simulink model "gofa_robot"  (R2023a)
settings: Solver=FixedStepAuto  StartTime=0.0  StopTime=11  FixedStep=0.001  RelTol=1e-3
undefined symbols (not defined in the file or in its folder): X, Y, Z
libraries: sm_lib x58, nesl_utility x10, slpidlib x3
(part 7 of 7)

== matlab function gofa_robot/inverse_Jacobian1 ==
  data: output_djoint_value output; dx input; det_J output; dy input; dz input; d_alpha input; d_beta input; d_gamma input; joint_value input
% function [dq1,dq2,dq3,dq4,dq5,dq6] = fcn(dx,dy,dz,d_alpha,d_beta,d_gamma, joint_value)
%function [output_joint_value,output_djoint_value,det_J]  = inverse_Jacobian(dx,dy,dz,d_alpha,d_beta,d_gamma, joint_value)
function [output_djoint_value,det_J]  = inverse_Jacobian(dx,dy,dz,d_alpha,d_beta,d_gamma, joint_value)
% persistent theta1 theta2 theta3 theta4 theta5 theta6
% if isempty(theta1)
%     theta1 =  1e-5;
%     theta2 =  1e-5;
%     theta3 =  1e-5;
%     theta4 =  1e-5;
%     theta5 =  1e-5;
%     theta6 =  1e-5;    
% end

if (length(joint_value)>1)
    q1 = joint_value(1);
    q2 = joint_value(2);
    q3 = joint_value(3);
    q4 = joint_value(4);
    q5 = joint_value(5);
    q6 = joint_value(6);
else
    q1 =  1e-5;
    q2 =  1e-5;
    q3 =  1e-5;
    q4 =  1e-5;
    q5 =  1e-5;
    q6 =  1e-5;
end

J = zeros(6,6);
J(1,1)= (551421093602387721*cos(q1)*cos(q2))/20282409603651670423947251286016000 - (15367999408544611283610854417045082301222635242944759808457209068371609267073198931*cos(q1))/533996758980227520598755426542388028650676130589163192486760401955554931445160137505740521734144000 - (501743517602172611*cos(q1)*cos(q4))/81129638414606681695789005144064000 + (3093548567763867359251342063207821441907716257110899757329320000341*sin(q3)*((81129638414606676728031405122553*cos(q1 - q2))/2 - (81129638414606686663546605165575*cos(q1 + q2))/2))/533996758980227520598755426542388028650676130589163192486760401955554931445160137505740521734144000 - (3093548567763867359251342063207821441907716257110899757329320000341*cos(q3)*((81129638414606676728031405122553*sin(q1 - q2))/2 + (81129638414606686663546605165575*sin(q1 + q2))/2))/533996758980227520598755426542388028650676130589163192486760401955554931445160137505740521734144000 - (111*sin(q1)*sin(q2))/250 - (11*sin(q3)*((81129638414606676728031405122553*sin(q1 - q2))/2 + (81129638414606686663546605165575*sin(q1 + q2))/2))/8112963841460668169578900514406400 - (101*cos(q5)*((81129638414606686663546605165575*sin(q1 + q2 + q3))/162259276829213363391578010288128 - (81129638414606676728031405122553*sin(q2 - q1 + q3))/162259276829213363391578010288128 + (4967757600021511*cos(q1))/81129638414606681695789005144064))/1000 - (sin(q5)*(81129638414606686663546605165575*sin(q1 + q2 + q3) - 81129638414606676728031405122553*sin(q2 - q1 + q3) + 9935515200043022*cos(q1)))/2028240960365167042394725128601600 - (501743517602172611*cos(q5)*((sin(q4)*(81129638414606686663546605165575*cos(q1 + q2 + q3) - 81129638414606676728031405122553*cos(q2 - q1 + q3)))/162259276829213363391578010288128 - cos(q1)*cos(q4) + (4967757600021511*cos(q4)*((81129638414606686663546605165575*sin(q1 + q2 + q3))/162259276829213363391578010288128 - (81129638414606676728031405122553*sin(q2 - q1 + q3))/162259276829213363391578010288128))/81129638414606681695789005144064))/81129638414606681695789005144064000 + (2*cos(q5)*(cos(q1)*sin(q4) - (4967757600021511*sin(q4)*((81129638414606686663546605165575*sin(q1 + q2 + q3))/162259276829213363391578010288128 - (81129638414606676728031405122553*sin(q2 - q1 + q3))/162259276829213363391578010288128))/81129638414606681695789005144064 + cos(q4)*((81129638414606686663546605165575*cos(q1 + q2 + q3))/162259276829213363391578010288128 - (81129638414606676728031405122553*cos(q2 - q1 + q3))/162259276829213363391578010288128)))/25 - (4967757600021511*sin(q5)*((sin(q4)*(81129638414606686663546605165575*cos(q1 + q2 + q3) - 81129638414606676728031405122553*cos(q2 - q1 + q3)))/162259276829213363391578010288128 - cos(q1)*cos(q4) + (4967757600021511*cos(q4)*((81129638414606686663546605165575*sin(q1 + q2 + q3))/162259276829213363391578010288128 - (81129638414606676728031405122553*sin(q2 - q1 + q3))/162259276829213363391578010288128))/81129638414606681695789005144064))/1014120480182583521197362564300800 - (101*sin(q5)*(cos(q1)*sin(q4) - (4967757600021511*sin(q4)*((81129638414606686663546605165575*sin(q1 + q2 + q3))/162259276829213363391578010288128 - (81129638414606676728031405122553*sin(q2 - q1 + q3))/162259276829213363391578010288128))/81129638414606681695789005144064 + cos(q4)*((81129638414606686663546605165575*cos(q1 + q2 + q3))/162259276829213363391578010288128 - (81129638414606676728031405122553*cos(q2 - q1 + q3))/162259276829213363391578010288128)))/1000 + (501743517602172611*sin(q4)*((81129638414606686663546605165575*cos(q1 + q2 + q3))/162259276829213363391578010288128 - (81129638414606676728031405122553*cos(q2 - q1 + q3))/162259276829213363391578010288128))/81129638414606681695789005144064000 - (11*cos(q3)*((81129638414606676728031405122553*cos(q1 - q2))/2 - (81129638414606686663546605165575*cos(q1 + q2))/2))/8112963841460668169578900514406400 + (2492540172829719769614233935035221*cos(q4)*((81129638414606686663546605165575*sin(q1 + q2 + q3))/162259276829213363391578010288128 - (81129638414606676728031405122553*sin(q2 - q1 + q3))/162259276829213363391578010288128))/6582018229284824168619876730229402019930943462534319453394436096000;
J(1,2)=(111*cos(q1)*cos(q2))/250 - (3093548567763867359251342063207821441907716257110899757329320000341*sin(q3)*((81129638414606676728031405122553*cos(q1 - q2))/2 + (81129638414606686663546605165575*cos(q1 + q2))/2))/533996758980227520598755426542388028650676130589163192486760401955554931445160137505740521734144000 - (sin(q5)*(81129638414606686663546605165575*sin(q1 + q2 + q3) + 81129638414606676728031405122553*sin(q2 - q1 + q3)))/2028240960365167042394725128601600 + (3093548567763867359251342063207821441907716257110899757329320000341*cos(q3)*((81129638414606676728031405122553*sin(q1 - q2))/2 - (81129638414606686663546605165575*sin(q1 + q2))/2))/533996758980227520598755426542388028650676130589163192486760401955554931445160137505740521734144000 - (551421093602387721*sin(q1)*sin(q2))/20282409603651670423947251286016000 + (11*sin(q3)*((81129638414606676728031405122553*sin(q1 - q2))/2 - (81129638414606686663546605165575*sin(q1 + q2))/2))/8112963841460668169578900514406400 - (501743517602172611*cos(q5)*(sin(q4)*((81129638414606686663546605165575*cos(q1 + q2 + q3))/162259276829213363391578010288128 + (81129638414606676728031405122553*cos(q2 - q1 + q3))/162259276829213363391578010288128) + (4967757600021511*cos(q4)*((81129638414606686663546605165575*sin(q1 + q2 + q3))/162259276829213363391578010288128 + (81129638414606676728031405122553*sin(q2 - q1 + q3))/162259276829213363391578010288128))/81129638414606681695789005144064))/81129638414606681695789005144064000 - (2*cos(q5)*((4967757600021511*sin(q4)*((81129638414606686663546605165575*sin(q1 + q2 + q3))/162259276829213363391578010288128 + (81129638414606676728031405122553*sin(q2 - q1 + q3))/162259276829213363391578010288128))/81129638414606681695789005144064 - cos(q4)*((81129638414606686663546605165575*cos(q1 + q2 + q3))/162259276829213363391578010288128 + (81129638414606676728031405122553*cos(q2 - q1 + q3))/162259276829213363391578010288128)))/25 - (4967757600021511*sin(q5)*(sin(q4)*((81129638414606686663546605165575*cos(q1 + q2 + q3))/162259276829213363391578010288128 + (81129638414606676728031405122553*cos(q2 - q1 + q3))/162259276829213363391578010288128) + (4967757600021511*cos(q4)*((81129638414606686663546605165575*sin(q1 + q2 + q3))/162259276829213363391578010288128 + (81129638414606676728031405122553*sin(q2 - q1 + q3))/162259276829213363391578010288128))/81129638414606681695789005144064))/1014120480182583521197362564300800 + (101*sin(q5)*((4967757600021511*sin(q4)*((81129638414606686663546605165575*sin(q1 + q2 + q3))/162259276829213363391578010288128 + (81129638414606676728031405122553*sin(q2 - q1 + q3))/162259276829213363391578010288128))/81129638414606681695789005144064 - cos(q4)*((81129638414606686663546605165575*cos(q1 + q2 + q3))/162259276829213363391578010288128 + (81129638414606676728031405122553*cos(q2 - q1 + q3))/162259276829213363391578010288128)))/1000 + (501743517602172611*sin(q4)*((81129638414606686663546605165575*cos(q1 + q2 + q3))/162259276829213363391578010288128 + (81129638414606676728031405122553*cos(q2 - q1 + q3))/162259276829213363391578010288128))/81129638414606681695789005144064000 + (11*cos(q3)*((81129638414606676728031405122553*cos(q1 - q2))/2 + (81129638414606686663546605165575*cos(q1 + q2))/2))/8112963841460668169578900514406400 + (2492540172829719769614233935035221*cos(q4)*((81129638414606686663546605165575*sin(q1 + q2 + q3))/162259276829213363391578010288128 + (81129638414606676728031405122553*sin(q2 - q1 + q3))/162259276829213363391578010288128))/6582018229284824168619876730229402019930943462534319453394436096000 - (101*cos(q5)*((81129638414606686663546605165575*sin(q1 + q2 + q3))/162259276829213363391578010288128 + (81129638414606676728031405122553*sin(q2 - q1 + q3))/162259276829213363391578010288128))/1000;
J(1,3)= (3093548567763867359251342063207821441907716257110899757329320000341*cos(q3)*((81129638414606676728031405122553*sin(q1 - q2))/2 - (81129638414606686663546605165575*sin(q1 + q2))/2))/533996758980227520598755426542388028650676130589163192486760401955554931445160137505740521734144000 - (sin(q5)*(81129638414606686663546605165575*sin(q1 + q2 + q3) + 81129638414606676728031405122553*sin(q2 - q1 + q3)))/2028240960365167042394725128601600 - (3093548567763867359251342063207821441907716257110899757329320000341*sin(q3)*((81129638414606676728031405122553*cos(q1 - q2))/2 + (81129638414606686663546605165575*cos(q1 + q2))/2))/533996758980227520598755426542388028650676130589163192486760401955554931445160137505740521734144000 + (11*sin(q3)*((81129638414606676728031405122553*sin(q1 - q2))/2 - (81129638414606686663546605165575*sin(q1 + q2))/2))/8112963841460668169578900514406400 - (501743517602172611*cos(q5)*(sin(q4)*((81129638414606686663546605165575*cos(q1 + q2 + q3))/162259276829213363391578010288128 + (81129638414606676728031405122553*cos(q2 - q1 + q3))/162259276829213363391578010288128) + (4967757600021511*cos(q4)*((81129638414606686663546605165575*sin(q1 + q2 + q3))/162259276829213363391578010288128 + (81129638414606676728031405122553*sin(q2 - q1 + q3))/162259276829213363391578010288128))/81129638414606681695789005144064))/81129638414606681695789005144064000 - (2*cos(q5)*((4967757600021511*sin(q4)*((81129638414606686663546605165575*sin(q1 + q2 + q3))/162259276829213363391578010288128 + (81129638414606676728031405122553*sin(q2 - q1 + q3))/162259276829213363391578010288128))/81129638414606681695789005144064 - cos(q4)*((81129638414606686663546605165575*cos(q1 + q2 + q3))/162259276829213363391578010288128 + (81129638414606676728031405122553*cos(q2 - q1 + q3))/162259276829213363391578010288128)))/25 - (4967757600021511*sin(q5)*(sin(q4)*((81129638414606686663546605165575*cos(q1 + q2 + q3))/162259276829213363391578010288128 + (81129638414606676728031405122553*cos(q2 - q1 + q3))/162259276829213363391578010288128) + (4967757600021511*cos(q4)*((81129638414606686663546605165575*sin(q1 + q2 + q3))/162259276829213363391578010288128 + (81129638414606676728031405122553*sin(q2 - q1 + q3))/162259276829213363391578010288128))/81129638414606681695789005144064))/1014120480182583521197362564300800 + (101*sin(q5)*((4967757600021511*sin(q4)*((81129638414606686663546605165575*sin(q1 + q2 + q3))/162259276829213363391578010288128 + (81129638414606676728031405122553*sin(q2 - q1 + q3))/162259276829213363391578010288128))/81129638414606681695789005144064 - cos(q4)*((81129638414606686663546605165575*cos(q1 + q2 + q3))/162259276829213363391578010288128 + (81129638414606676728031405122553*cos(q2 - q1 + q3))/162259276829213363391578010288128)))/1000 + (501743517602172611*sin(q4)*((81129638414606686663546605165575*cos(q1 + q2 + q3))/162259276829213363391578010288128 + (81129638414606676728031405122553*cos(q2 - q1 + q3))/162259276829213363391578010288128))/81129638414606681695789005144064000 + (11*cos(q3)*((81129638414606676728031405122553*cos(q1 - q2))/2 + (81129638414606686663546605165575*cos(q1 + q2))/2))/8112963841460668169578900514406400 + (2492540172829719769614233935035221*cos(q4)*((81129638414606686663546605165575*sin(q1 + q2 + q3))/162259276829213363391578010288128 + (81129638414606676728031405122553*sin(q2 - q1 + q3))/162259276829213363391578010288128))/6582018229284824168619876730229402019930943462534319453394436096000 - (101*cos(q5)*((81129638414606686663546605165575*sin(q1 + q2 + q3))/162259276829213363391578010288128 + (81129638414606676728031405122553*sin(q2 - q1 + q3))/162259276829213363391578010288128))/1000;
J(1,4)=(501743517602172611*sin(q1)*sin(q4))/81129638414606681695789005144064000 + (2*cos(q5)*(cos(q4)*sin(q1) - sin(q4)*((81129638414606686663546605165575*sin(q1 + q2 + q3))/162259276829213363391578010288128 + (81129638414606676728031405122553*sin(q2 - q1 + q3))/162259276829213363391578010288128) + (4967757600021511*cos(q4)*((81129638414606686663546605165575*cos(q1 + q2 + q3))/162259276829213363391578010288128 + (81129638414606676728031405122553*cos(q2 - q1 + q3))/162259276829213363391578010288128))/81129638414606681695789005144064))/25 - (501743517602172611*cos(q5)*(sin(q1)*sin(q4) + (4967757600021511*sin(q4)*((81129638414606686663546605165575*cos(q1 + q2 + q3))/162259276829213363391578010288128 + (81129638414606676728031405122553*cos(q2 - q1 + q3))/162259276829213363391578010288128))/81129638414606681695789005144064 + cos(q4)*((81129638414606686663546605165575*sin(q1 + q2 + q3))/162259276829213363391578010288128 + (81129638414606676728031405122553*sin(q2 - q1 + q3))/162259276829213363391578010288128)))/81129638414606681695789005144064000 - (101*sin(q5)*(cos(q4)*sin(q1) - sin(q4)*((81129638414606686663546605165575*sin(q1 + q2 + q3))/162259276829213363391578010288128 + (81129638414606676728031405122553*sin(q2 - q1 + q3))/162259276829213363391578010288128) + (4967757600021511*cos(q4)*((81129638414606686663546605165575*cos(q1 + q2 + q3))/162259276829213363391578010288128 + (81129638414606676728031405122553*cos(q2 - q1 + q3))/162259276829213363391578010288128))/81129638414606681695789005144064))/1000 - (4967757600021511*sin(q5)*(sin(q1)*sin(q4) + (4967757600021511*sin(q4)*((81129638414606686663546605165575*cos(q1 + q2 + q3))/162259276829213363391578010288128 + (81129638414606676728031405122553*cos(q2 - q1 + q3))/162259276829213363391578010288128))/81129638414606681695789005144064 + cos(q4)*((81129638414606686663546605165575*sin(q1 + q2 + q3))/162259276829213363391578010288128 + (81129638414606676728031405122553*sin(q2 - q1 + q3))/162259276829213363391578010288128)))/1014120480182583521197362564300800 + (2492540172829719769614233935035221*sin(q4)*((81129638414606686663546605165575*cos(q1 + q2 + q3))/162259276829213363391578010288128 + (81129638414606676728031405122553*cos(q2 - q1 + q3))/162259276829213363391578010288128))/6582018229284824168619876730229402019930943462534319453394436096000 + (501743517602172611*cos(q4)*((81129638414606686663546605165575*sin(q1 + q2 + q3))/162259276829213363391578010288128 + (81129638414606676728031405122553*sin(q2 - q1 + q3))/162259276829213363391578010288128))/81129638414606681695789005144064000;
J(1,5)=(cos(q5)*(81129638414606686663546605165575*cos(q1 + q2 + q3) + 81129638414606676728031405122553*cos(q2 - q1 + q3) - 9935515200043022*sin(q1)))/2028240960365167042394725128601600 - (101*sin(q5)*((81129638414606686663546605165575*cos(q1 + q2 + q3))/162259276829213363391578010288128 + (81129638414606676728031405122553*cos(q2 - q1 + q3))/162259276829213363391578010288128 - (4967757600021511*sin(q1))/81129638414606681695789005144064))/1000 + (4967757600021511*cos(q5)*(cos(q4)*sin(q1) - sin(q4)*((81129638414606686663546605165575*sin(q1 + q2 + q3))/162259276829213363391578010288128 + (81129638414606676728031405122553*sin(q2 - q1 + q3))/162259276829213363391578010288128) + (4967757600021511*cos(q4)*((81129638414606686663546605165575*cos(q1 + q2 + q3))/162259276829213363391578010288128 + (81129638414606676728031405122553*cos(q2 - q1 + q3))/162259276829213363391578010288128))/81129638414606681695789005144064))/1014120480182583521197362564300800 - (101*cos(q5)*(sin(q1)*sin(q4) + (4967757600021511*sin(q4)*((81129638414606686663546605165575*cos(q1 + q2 + q3))/162259276829213363391578010288128 + (81129638414606676728031405122553*cos(q2 - q1 + q3))/162259276829213363391578010288128))/81129638414606681695789005144064 + cos(q4)*((81129638414606686663546605165575*sin(q1 + q2 + q3))/162259276829213363391578010288128 + (81129638414606676728031405122553*sin(q2 - q1 + q3))/162259276829213363391578010288128)))/1000 - (501743517602172611*sin(q5)*(cos(q4)*sin(q1) - sin(q4)*((81129638414606686663546605165575*sin(q1 + q2 + q3))/162259276829213363391578010288128 + (81129638414606676728031405122553*sin(q2 - q1 + q3))/162259276829213363391578010288128) + (4967757600021511*cos(q4)*((81129638414606686663546605165575*cos(q1 + q2 + q3))/162259276829213363391578010288128 + (81129638414606676728031405122553*cos(q2 - q1 + q3))/162259276829213363391578010288128))/81129638414606681695789005144064))/81129638414606681695789005144064000 - (2*sin(q5)*(sin(q1)*sin(q4) + (4967757600021511*sin(q4)*((81129638414606686663546605165575*cos(q1 + q2 + q3))/162259276829213363391578010288128 + (81129638414606676728031405122553*cos(q2 - q1 + q3))/162259276829213363391578010288128))/81129638414606681695789005144064 + cos(q4)*((81129638414606686663546605165575*sin(q1 + q2 + q3))/162259276829213363391578010288128 + (81129638414606676728031405122553*sin(q2 - q1 + q3))/162259276829213363391578010288128)))/25;
J(1,6)= 0;

J(2,1)=(11*sin(q3)*((81129638414606676728031405122553*cos(q1 - q2))/2 + (81129638414606686663546605165575*cos(q1 + q2))/2))/8112963841460668169578900514406400 - (15367999408544611283610854417045082301222635242944759808457209068371609267073198931*sin(q1))/533996758980227520598755426542388028650676130589163192486760401955554931445160137505740521734144000 + (501743517602172611*sin(q4)*((81129638414606686663546605165575*sin(q1 + q2 + q3))/162259276829213363391578010288128 + (81129638414606676728031405122553*sin(q2 - q1 + q3))/162259276829213363391578010288128))/81129638414606681695789005144064000 + (111*cos(q1)*sin(q2))/250 + (551421093602387721*cos(q2)*sin(q1))/20282409603651670423947251286016000 - (501743517602172611*cos(q4)*sin(q1))/81129638414606681695789005144064000 - (11*cos(q3)*((81129638414606676728031405122553*sin(q1 - q2))/2 - (81129638414606686663546605165575*sin(q1 + q2))/2))/8112963841460668169578900514406400 + (3093548567763867359251342063207821441907716257110899757329320000341*sin(q3)*((81129638414606676728031405122553*sin(q1 - q2))/2 - (81129638414606686663546605165575*sin(q1 + q2))/2))/533996758980227520598755426542388028650676130589163192486760401955554931445160137505740521734144000 + (101*cos(q5)*((81129638414606686663546605165575*cos(q1 + q2 + q3))/162259276829213363391578010288128 + (81129638414606676728031405122553*cos(q2 - q1 + q3))/162259276829213363391578010288128 - (4967757600021511*sin(q1))/81129638414606681695789005144064))/1000 + (sin(q5)*(81129638414606686663546605165575*cos(q1 + q2 + q3) + 81129638414606676728031405122553*cos(q2 - q1 + q3) - 9935515200043022*sin(q1)))/2028240960365167042394725128601600 + (501743517602172611*cos(q5)*(cos(q4)*sin(q1) - sin(q4)*((81129638414606686663546605165575*sin(q1 + q2 + q3))/162259276829213363391578010288128 + (81129638414606676728031405122553*sin(q2 - q1 + q3))/162259276829213363391578010288128) + (4967757600021511*cos(q4)*((81129638414606686663546605165575*cos(q1 + q2 + q3))/162259276829213363391578010288128 + (81129638414606676728031405122553*cos(q2 - q1 + q3))/162259276829213363391578010288128))/81129638414606681695789005144064))/81129638414606681695789005144064000 + (2*cos(q5)*(sin(q1)*sin(q4) + (4967757600021511*sin(q4)*((81129638414606686663546605165575*cos(q1 + q2 + q3))/162259276829213363391578010288128 + (81129638414606676728031405122553*cos(q2 - q1 + q3))/162259276829213363391578010288128))/81129638414606681695789005144064 + cos(q4)*((81129638414606686663546605165575*sin(q1 + q2 + q3))/162259276829213363391578010288128 + (81129638414606676728031405122553*sin(q2 - q1 + q3))/162259276829213363391578010288128)))/25 + (4967757600021511*sin(q5)*(cos(q4)*sin(q1) - sin(q4)*((81129638414606686663546605165575*sin(q1 + q2 + q3))/162259276829213363391578010288128 + (81129638414606676728031405122553*sin(q2 - q1 + q3))/162259276829213363391578010288128) + (4967757600021511*cos(q4)*((81129638414606686663546605165575*cos(q1 + q2 + q3))/162259276829213363391578010288128 + (81129638414606676728031405122553*cos(q2 - q1 + q3))/162259276829213363391578010288128))/81129638414606681695789005144064))/1014120480182583521197362564300800 - (2492540172829719769614233935035221*cos(q4)*((81129638414606686663546605165575*cos(q1 + q2 + q3))/162259276829213363391578010288128 + (81129638414606676728031405122553*cos(q2 - q1 + q3))/162259276829213363391578010288128))/6582018229284824168619876730229402019930943462534319453394436096000 - (101*sin(q5)*(sin(q1)*sin(q4) + (4967757600021511*sin(q4)*((81129638414606686663546605165575*cos(q1 + q2 + q3))/162259276829213363391578010288128 + (81129638414606676728031405122553*cos(q2 - q1 + q3))/162259276829213363391578010288128))/81129638414606681695789005144064 + cos(q4)*((81129638414606686663546605165575*sin(q1 + q2 + q3))/162259276829213363391578010288128 + (81129638414606676728031405122553*sin(q2 - q1 + q3))/162259276829213363391578010288128)))/1000 + (3093548567763867359251342063207821441907716257110899757329320000341*cos(q3)*((81129638414606676728031405122553*cos(q1 - q2))/2 + (81129638414606686663546605165575*cos(q1 + q2))/2))/533996758980227520598755426542388028650676130589163192486760401955554931445160137505740521734144000;
J(2,2)=(501743517602172611*sin(q4)*((81129638414606686663546605165575*sin(q1 + q2 + q3))/162259276829213363391578010288128 - (81129638414606676728031405122553*sin(q2 - q1 + q3))/162259276829213363391578010288128))/81129638414606681695789005144064000 - (11*sin(q3)*((81129638414606676728031405122553*cos(q1 - q2))/2 - (81129638414606686663546605165575*cos(q1 + q2))/2))/8112963841460668169578900514406400 + (551421093602387721*cos(q1)*sin(q2))/20282409603651670423947251286016000 + (111*cos(q2)*sin(q1))/250 + (11*cos(q3)*((81129638414606676728031405122553*sin(q1 - q2))/2 + (81129638414606686663546605165575*sin(q1 + q2))/2))/8112963841460668169578900514406400 - (3093548567763867359251342063207821441907716257110899757329320000341*sin(q3)*((81129638414606676728031405122553*sin(q1 - q2))/2 + (81129638414606686663546605165575*sin(q1 + q2))/2))/533996758980227520598755426542388028650676130589163192486760401955554931445160137505740521734144000 - (501743517602172611*cos(q5)*((sin(q4)*(81129638414606686663546605165575*sin(q1 + q2 + q3) - 81129638414606676728031405122553*sin(q2 - q1 + q3)))/162259276829213363391578010288128 - (4967757600021511*cos(q4)*((81129638414606686663546605165575*cos(q1 + q2 + q3))/162259276829213363391578010288128 - (81129638414606676728031405122553*cos(q2 - q1 + q3))/162259276829213363391578010288128))/81129638414606681695789005144064))/81129638414606681695789005144064000 + (2*cos(q5)*((4967757600021511*sin(q4)*((81129638414606686663546605165575*cos(q1 + q2 + q3))/162259276829213363391578010288128 - (81129638414606676728031405122553*cos(q2 - q1 + q3))/162259276829213363391578010288128))/81129638414606681695789005144064 + (cos(q4)*(81129638414606686663546605165575*sin(q1 + q2 + q3) - 81129638414606676728031405122553*sin(q2 - q1 + q3)))/162259276829213363391578010288128))/25 - (4967757600021511*sin(q5)*((sin(q4)*(81129638414606686663546605165575*sin(q1 + q2 + q3) - 81129638414606676728031405122553*sin(q2 - q1 + q3)))/162259276829213363391578010288128 - (4967757600021511*cos(q4)*((81129638414606686663546605165575*cos(q1 + q2 + q3))/162259276829213363391578010288128 - (81129638414606676728031405122553*cos(q2 - q1 + q3))/162259276829213363391578010288128))/81129638414606681695789005144064))/1014120480182583521197362564300800 - (101*sin(q5)*((4967757600021511*sin(q4)*((81129638414606686663546605165575*cos(q1 + q2 + q3))/162259276829213363391578010288128 - (81129638414606676728031405122553*cos(q2 - q1 + q3))/162259276829213363391578010288128))/81129638414606681695789005144064 + (cos(q4)*(81129638414606686663546605165575*sin(q1 + q2 + q3) - 81129638414606676728031405122553*sin(q2 - q1 + q3)))/162259276829213363391578010288128))/1000 - (2492540172829719769614233935035221*cos(q4)*((81129638414606686663546605165575*cos(q1 + q2 + q3))/162259276829213363391578010288128 - (81129638414606676728031405122553*cos(q2 - q1 + q3))/162259276829213363391578010288128))/6582018229284824168619876730229402019930943462534319453394436096000 + (101*cos(q5)*((81129638414606686663546605165575*cos(q1 + q2 + q3))/162259276829213363391578010288128 - (81129638414606676728031405122553*cos(q2 - q1 + q3))/162259276829213363391578010288128))/1000 + (sin(q5)*(81129638414606686663546605165575*cos(q1 + q2 + q3) - 81129638414606676728031405122553*cos(q2 - q1 + q3)))/2028240960365167042394725128601600 - (3093548567763867359251342063207821441907716257110899757329320000341*cos(q3)*((81129638414606676728031405122553*cos(q1 - q2))/2 - (81129638414606686663546605165575*cos(q1 + q2))/2))/533996758980227520598755426542388028650676130589163192486760401955554931445160137505740521734144000;
J(2,3)=(501743517602172611*sin(q4)*((81129638414606686663546605165575*sin(q1 + q2 + q3))/162259276829213363391578010288128 - (81129638414606676728031405122553*sin(q2 - q1 + q3))/162259276829213363391578010288128))/81129638414606681695789005144064000 - (11*sin(q3)*((81129638414606676728031405122553*cos(q1 - q2))/2 - (81129638414606686663546605165575*cos(q1 + q2))/2))/8112963841460668169578900514406400 + (11*cos(q3)*((81129638414606676728031405122553*sin(q1 - q2))/2 + (81129638414606686663546605165575*sin(q1 + q2))/2))/8112963841460668169578900514406400 - (3093548567763867359251342063207821441907716257110899757329320000341*sin(q3)*((81129638414606676728031405122553*sin(q1 - q2))/2 + (81129638414606686663546605165575*sin(q1 + q2))/2))/533996758980227520598755426542388028650676130589163192486760401955554931445160137505740521734144000 - (501743517602172611*cos(q5)*((sin(q4)*(81129638414606686663546605165575*sin(q1 + q2 + q3) - 81129638414606676728031405122553*sin(q2 - q1 + q3)))/162259276829213363391578010288128 - (4967757600021511*cos(q4)*((81129638414606686663546605165575*cos(q1 + q2 + q3))/162259276829213363391578010288128 - (81129638414606676728031405122553*cos(q2 - q1 + q3))/162259276829213363391578010288128))/81129638414606681695789005144064))/81129638414606681695789005144064000 + (2*cos(q5)*((4967757600021511*sin(q4)*((81129638414606686663546605165575*cos(q1 + q2 + q3))/162259276829213363391578010288128 - (81129638414606676728031405122553*cos(q2 - q1 + q3))/162259276829213363391578010288128))/81129638414606681695789005144064 + (cos(q4)*(81129638414606686663546605165575*sin(q1 + q2 + q3) - 81129638414606676728031405122553*sin(q2 - q1 + q3)))/162259276829213363391578010288128))/25 - (4967757600021511*sin(q5)*((sin(q4)*(81129638414606686663546605165575*sin(q1 + q2 + q3) - 81129638414606676728031405122553*sin(q2 - q1 + q3)))/162259276829213363391578010288128 - (4967757600021511*cos(q4)*((81129638414606686663546605165575*cos(q1 + q2 + q3))/162259276829213363391578010288128 - (81129638414606676728031405122553*cos(q2 - q1 + q3))/162259276829213363391578010288128))/81129638414606681695789005144064))/1014120480182583521197362564300800 - (101*sin(q5)*((4967757600021511*sin(q4)*((81129638414606686663546605165575*cos(q1 + q2 + q3))/162259276829213363391578010288128 - (81129638414606676728031405122553*cos(q2 - q1 + q3))/162259276829213363391578010288128))/81129638414606681695789005144064 + (cos(q4)*(81129638414606686663546605165575*sin(q1 + q2 + q3) - 81129638414606676728031405122553*sin(q2 - q1 + q3)))/162259276829213363391578010288128))/1000 - (2492540172829719769614233935035221*cos(q4)*((81129638414606686663546605165575*cos(q1 + q2 + q3))/162259276829213363391578010288128 - (81129638414606676728031405122553*cos(q2 - q1 + q3))/162259276829213363391578010288128))/6582018229284824168619876730229402019930943462534319453394436096000 + (101*cos(q5)*((81129638414606686663546605165575*cos(q1 + q2 + q3))/162259276829213363391578010288128 - (81129638414606676728031405122553*cos(q2 - q1 + q3))/162259276829213363391578010288128))/1000 + (sin(q5)*(81129638414606686663546605165575*cos(q1 + q2 + q3) - 81129638414606676728031405122553*cos(q2 - q1 + q3)))/2028240960365167042394725128601600 - (3093548567763867359251342063207821441907716257110899757329320000341*cos(q3)*((81129638414606676728031405122553*cos(q1 - q2))/2 - (81129638414606686663546605165575*cos(q1 + q2))/2))/533996758980227520598755426542388028650676130589163192486760401955554931445160137505740521734144000;
J(2,4)=(2492540172829719769614233935035221*sin(q4)*((81129638414606686663546605165575*sin(q1 + q2 + q3))/162259276829213363391578010288128 - (81129638414606676728031405122553*sin(q2 - q1 + q3))/162259276829213363391578010288128))/6582018229284824168619876730229402019930943462534319453394436096000 - (501743517602172611*cos(q1)*sin(q4))/81129638414606681695789005144064000 + (2*cos(q5)*((sin(q4)*(81129638414606686663546605165575*cos(q1 + q2 + q3) - 81129638414606676728031405122553*cos(q2 - q1 + q3)))/162259276829213363391578010288128 - cos(q1)*cos(q4) + (4967757600021511*cos(q4)*((81129638414606686663546605165575*sin(q1 + q2 + q3))/162259276829213363391578010288128 - (81129638414606676728031405122553*sin(q2 - q1 + q3))/162259276829213363391578010288128))/81129638414606681695789005144064))/25 + (501743517602172611*cos(q5)*(cos(q1)*sin(q4) - (4967757600021511*sin(q4)*((81129638414606686663546605165575*sin(q1 + q2 + q3))/162259276829213363391578010288128 - (81129638414606676728031405122553*sin(q2 - q1 + q3))/162259276829213363391578010288128))/81129638414606681695789005144064 + cos(q4)*((81129638414606686663546605165575*cos(q1 + q2 + q3))/162259276829213363391578010288128 - (81129638414606676728031405122553*cos(q2 - q1 + q3))/162259276829213363391578010288128)))/81129638414606681695789005144064000 - (101*sin(q5)*((sin(q4)*(81129638414606686663546605165575*cos(q1 + q2 + q3) - 81129638414606676728031405122553*cos(q2 - q1 + q3)))/162259276829213363391578010288128 - cos(q1)*cos(q4) + (4967757600021511*cos(q4)*((81129638414606686663546605165575*sin(q1 + q2 + q3))/162259276829213363391578010288128 - (81129638414606676728031405122553*sin(q2 - q1 + q3))/162259276829213363391578010288128))/81129638414606681695789005144064))/1000 + (4967757600021511*sin(q5)*(cos(q1)*sin(q4) - (4967757600021511*sin(q4)*((81129638414606686663546605165575*sin(q1 + q2 + q3))/162259276829213363391578010288128 - (81129638414606676728031405122553*sin(q2 - q1 + q3))/162259276829213363391578010288128))/81129638414606681695789005144064 + cos(q4)*((81129638414606686663546605165575*cos(q1 + q2 + q3))/162259276829213363391578010288128 - (81129638414606676728031405122553*cos(q2 - q1 + q3))/162259276829213363391578010288128)))/1014120480182583521197362564300800 - (501743517602172611*cos(q4)*((81129638414606686663546605165575*cos(q1 + q2 + q3))/162259276829213363391578010288128 - (81129638414606676728031405122553*cos(q2 - q1 + q3))/162259276829213363391578010288128))/81129638414606681695789005144064000;
J(2,5)=(cos(q5)*(81129638414606686663546605165575*sin(q1 + q2 + q3) - 81129638414606676728031405122553*sin(q2 - q1 + q3) + 9935515200043022*cos(q1)))/2028240960365167042394725128601600 - (101*sin(q5)*((81129638414606686663546605165575*sin(q1 + q2 + q3))/162259276829213363391578010288128 - (81129638414606676728031405122553*sin(q2 - q1 + q3))/162259276829213363391578010288128 + (4967757600021511*cos(q1))/81129638414606681695789005144064))/1000 + (4967757600021511*cos(q5)*((sin(q4)*(81129638414606686663546605165575*cos(q1 + q2 + q3) - 81129638414606676728031405122553*cos(q2 - q1 + q3)))/162259276829213363391578010288128 - cos(q1)*cos(q4) + (4967757600021511*cos(q4)*((81129638414606686663546605165575*sin(q1 + q2 + q3))/162259276829213363391578010288128 - (81129638414606676728031405122553*sin(q2 - q1 + q3))/162259276829213363391578010288128))/81129638414606681695789005144064))/1014120480182583521197362564300800 + (101*cos(q5)*(cos(q1)*sin(q4) - (4967757600021511*sin(q4)*((81129638414606686663546605165575*sin(q1 + q2 + q3))/162259276829213363391578010288128 - (81129638414606676728031405122553*sin(q2 - q1 + q3))/162259276829213363391578010288128))/81129638414606681695789005144064 + cos(q4)*((81129638414606686663546605165575*cos(q1 + q2 + q3))/162259276829213363391578010288128 - (81129638414606676728031405122553*cos(q2 - q1 + q3))/162259276829213363391578010288128)))/1000 - (501743517602172611*sin(q5)*((sin(q4)*(81129638414606686663546605165575*cos(q1 + q2 + q3) - 81129638414606676728031405122553*cos(q2 - q1 + q3)))/162259276829213363391578010288128 - cos(q1)*cos(q4) + (4967757600021511*cos(q4)*((81129638414606686663546605165575*sin(q1 + q2 + q3))/162259276829213363391578010288128 - (81129638414606676728031405122553*sin(q2 - q1 + q3))/162259276829213363391578010288128))/81129638414606681695789005144064))/81129638414606681695789005144064000 + (2*sin(q5)*(cos(q1)*sin(q4) - (4967757600021511*sin(q4)*((81129638414606686663546605165575*sin(q1 + q2 + q3))/162259276829213363391578010288128 - (81129638414606676728031405122553*sin(q2 - q1 + q3))/162259276829213363391578010288128))/81129638414606681695789005144064 + cos(q4)*((81129638414606686663546605165575*cos(q1 + q2 + q3))/162259276829213363391578010288128 - (81129638414606676728031405122553*cos(q2 - q1 + q3))/162259276829213363391578010288128)))/25;
J(2,6)= 0 ;

J(3,1)= 0;
J(3,2)= (1628250806397484373275779136617308223200615402653*cos(q2 + q3 + q4))/526561458342785933489590138418352161594475477002745556271554887680 - (40706270159937104346814132755993166351547514995883*cos(q2 + q3 - q4))/13164036458569648337239753460458804039861886925068638906788872192000 - (111*sin(q2))/250 - (52656145834278599797477058980386992099945290365275866185320645*16601^(1/2)*cos(q2 + q3 + q4 + q5 - atan(80/101)))/210624583337114373395836055367340864637790190801098222508621955072 + (263280729171392966744795069209175093652614835642058079429268519*16601^(1/2)*cos(q2 + q3 + q4 - q5 + atan(80/101)))/1053122916685571866979180276836704323188950954005491112543109775360 - (6582018229284823362555121087910479384599870772374890568949237809*16601^(1/2)*cos(q2 + q3 - q4 + q5 - atan(80/101)))/26328072917139296674479506920917608079723773850137277813577744384000 + (263280729171392966744795069209175093652614835642058079429268519*16601^(1/2)*cos(q2 + q3 - q4 - q5 + atan(80/101)))/1053122916685571866979180276836704323188950954005491112543109775360 - (16601^(1/2)*cos(q2 + q3 + q5 - atan(80/101)))/2000 - (16601^(1/2)*cos(q2 + q3 - q5 + atan(80/101)))/2000 - (10094250605158591598152664139145929529411442230104098116990665870556795300108196123912610710424694202051282578230955659697511666829881^(1/2)*cos(q2 + q3 - atan(724022005221330658548186440325234222192403780878775139873387970560/3093548567763867359251342063207821441907716257110899757329320000341)))/6582018229284824168619876730229402019930943462534319453394436096000;
J(3,3)= (1628250806397484373275779136617308223200615402653*cos(q2 + q3 + q4))/526561458342785933489590138418352161594475477002745556271554887680 - (40706270159937104346814132755993166351547514995883*cos(q2 + q3 - q4))/13164036458569648337239753460458804039861886925068638906788872192000 - (52656145834278599797477058980386992099945290365275866185320645*16601^(1/2)*cos(q2 + q3 + q4 + q5 - atan(80/101)))/210624583337114373395836055367340864637790190801098222508621955072 + (263280729171392966744795069209175093652614835642058079429268519*16601^(1/2)*cos(q2 + q3 + q4 - q5 + atan(80/101)))/1053122916685571866979180276836704323188950954005491112543109775360 - (6582018229284823362555121087910479384599870772374890568949237809*16601^(1/2)*cos(q2 + q3 - q4 + q5 - atan(80/101)))/26328072917139296674479506920917608079723773850137277813577744384000 + (263280729171392966744795069209175093652614835642058079429268519*16601^(1/2)*cos(q2 + q3 - q4 - q5 + atan(80/101)))/1053122916685571866979180276836704323188950954005491112543109775360 - (16601^(1/2)*cos(q2 + q3 + q5 - atan(80/101)))/2000 - (16601^(1/2)*cos(q2 + q3 - q5 + atan(80/101)))/2000 - (10094250605158591598152664139145929529411442230104098116990665870556795300108196123912610710424694202051282578230955659697511666829881^(1/2)*cos(q2 + q3 - atan(724022005221330658548186440325234222192403780878775139873387970560/3093548567763867359251342063207821441907716257110899757329320000341)))/6582018229284824168619876730229402019930943462534319453394436096000;
J(3,4)= (1628250806397484373275779136617308223200615402653*cos(q2 + q3 + q4))/526561458342785933489590138418352161594475477002745556271554887680 + (40706270159937104346814132755993166351547514995883*cos(q2 + q3 - q4))/13164036458569648337239753460458804039861886925068638906788872192000 - (2492540172829719769614233935035221*sin(q4))/6582018229284824168619876730229402019930943462534319453394436096000 - (52656145834278599797477058980386992099945290365275866185320645*16601^(1/2)*cos(q2 + q3 + q4 + q5 - atan(80/101)))/210624583337114373395836055367340864637790190801098222508621955072 + (263280729171392966744795069209175093652614835642058079429268519*16601^(1/2)*cos(q2 + q3 + q4 - q5 + atan(80/101)))/1053122916685571866979180276836704323188950954005491112543109775360 - (403032377821159448978357750059338280708391237583*16601^(1/2)*cos(q5 - q4 + atan(101/80)))/13164036458569648337239753460458804039861886925068638906788872192000 + (6582018229284823362555121087910479384599870772374890568949237809*16601^(1/2)*cos(q2 + q3 - q4 + q5 - atan(80/101)))/26328072917139296674479506920917608079723773850137277813577744384000 - (263280729171392966744795069209175093652614835642058079429268519*16601^(1/2)*cos(q2 + q3 - q4 - q5 + atan(80/101)))/1053122916685571866979180276836704323188950954005491112543109775360 - (16121295112846379933423555808092160625748667353*16601^(1/2)*cos(q4 + q5 + atan(101/80)))/526561458342785933489590138418352161594475477002745556271554887680;
J(3,5)= (403032377821159448978357750059338280708391237583*16601^(1/2)*cos(q5 - q4 + atan(101/80)))/13164036458569648337239753460458804039861886925068638906788872192000 - (263280729171392966744795069209175093652614835642058079429268519*16601^(1/2)*cos(q2 + q3 + q4 - q5 + atan(80/101)))/1053122916685571866979180276836704323188950954005491112543109775360 - (52656145834278599797477058980386992099945290365275866185320645*16601^(1/2)*cos(q2 + q3 + q4 + q5 - atan(80/101)))/210624583337114373395836055367340864637790190801098222508621955072 + (24678615572571482867467662723121*16601^(1/2)*cos(q5 + atan(101/80)))/6582018229284824168619876730229402019930943462534319453394436096000 - (6582018229284823362555121087910479384599870772374890568949237809*16601^(1/2)*cos(q2 + q3 - q4 + q5 - atan(80/101)))/26328072917139296674479506920917608079723773850137277813577744384000 - (263280729171392966744795069209175093652614835642058079429268519*16601^(1/2)*cos(q2 + q3 - q4 - q5 + atan(80/101)))/1053122916685571866979180276836704323188950954005491112543109775360 - (16601^(1/2)*cos(q2 + q3 + q5 - atan(80/101)))/2000 + (16601^(1/2)*cos(q2 + q3 - q5 + atan(80/101)))/2000 - (16121295112846379933423555808092160625748667353*16601^(1/2)*cos(q4 + q5 + atan(101/80)))/526561458342785933489590138418352161594475477002745556271554887680;
J(3,6)= 0;

J(4,1)= 0;
J(4,2)= -sin(q1);
J(4,3)= -sin(q1);
J(4,4)= (81129638414606686663546605165575*cos(q1 + q2 + q3))/162259276829213363391578010288128 + (81129638414606676728031405122553*cos(q2 - q1 + q3))/162259276829213363391578010288128 - (4967757600021511*sin(q1))/81129638414606681695789005144064; 
J(4,5)= (403032377821159498335588895202304015643716683825*cos(q1 + q2 + q3))/13164036458569648337239753460458804039861886925068638906788872192 - sin(q1 - q4)/2 + (6582018229284823362555121087910479384599870772374890568949237809*cos(q1 - q2 - q3 + q4))/26328072917139296674479506920917608079723773850137277813577744384 + (403032377821159448978357750059338280708391237583*cos(q2 - q1 + q3))/13164036458569648337239753460458804039861886925068638906788872192 - (6582018229284824974684632372548374012493161295659483273165080625*cos(q1 + q2 + q3 + q4))/26328072917139296674479506920917608079723773850137277813577744384 - sin(q1 + q4)/2 - (24678615572571482867467662723121*sin(q1))/6582018229284824168619876730229402019930943462534319453394436096 + (6582018229284824168619876730229377341315370891051451985731712975*cos(q1 + q2 + q3 - q4))/26328072917139296674479506920917608079723773850137277813577744384 - (6582018229284824168619876730229377341315370891051451985731712975*cos(q2 - q1 + q3 + q4))/26328072917139296674479506920917608079723773850137277813577744384;
J(4,6)= (4967757600021511*sin(q4)*((81129638414606686663546605165575*sin(q1 + q2 + q3))/162259276829213363391578010288128 + (81129638414606676728031405122553*sin(q2 - q1 + q3))/162259276829213363391578010288128))/81129638414606681695789005144064 - (122597380068651197257713859414983140362437055831*sin(q1))/533996758980227520598755426542388028650676130589163192486760401955554931445160137505740521734144 - (4967757600021511*cos(q4)*sin(q1))/81129638414606681695789005144064 + (24678615572571482867467662723121*sin(q3)*((81129638414606676728031405122553*sin(q1 - q2))/2 - (81129638414606686663546605165575*sin(q1 + q2))/2))/533996758980227520598755426542388028650676130589163192486760401955554931445160137505740521734144 + cos(q5)*((81129638414606686663546605165575*cos(q1 + q2 + q3))/162259276829213363391578010288128 + (81129638414606676728031405122553*cos(q2 - q1 + q3))/162259276829213363391578010288128 - (4967757600021511*sin(q1))/81129638414606681695789005144064) + (4967757600021511*cos(q5)*(cos(q4)*sin(q1) - sin(q4)*((81129638414606686663546605165575*sin(q1 + q2 + q3))/162259276829213363391578010288128 + (81129638414606676728031405122553*sin(q2 - q1 + q3))/162259276829213363391578010288128) + (4967757600021511*cos(q4)*((81129638414606686663546605165575*cos(q1 + q2 + q3))/162259276829213363391578010288128 + (81129638414606676728031405122553*cos(q2 - q1 + q3))/162259276829213363391578010288128))/81129638414606681695789005144064))/81129638414606681695789005144064 - (24678615572571482867467662723121*cos(q4)*((81129638414606686663546605165575*cos(q1 + q2 + q3))/162259276829213363391578010288128 + (81129638414606676728031405122553*cos(q2 - q1 + q3))/162259276829213363391578010288128))/6582018229284824168619876730229402019930943462534319453394436096 - sin(q5)*(sin(q1)*sin(q4) + (4967757600021511*sin(q4)*((81129638414606686663546605165575*cos(q1 + q2 + q3))/162259276829213363391578010288128 + (81129638414606676728031405122553*cos(q2 - q1 + q3))/162259276829213363391578010288128))/81129638414606681695789005144064 + cos(q4)*((81129638414606686663546605165575*sin(q1 + q2 + q3))/162259276829213363391578010288128 + (81129638414606676728031405122553*sin(q2 - q1 + q3))/162259276829213363391578010288128)) + (24678615572571482867467662723121*cos(q3)*((81129638414606676728031405122553*cos(q1 - q2))/2 + (81129638414606686663546605165575*cos(q1 + q2))/2))/533996758980227520598755426542388028650676130589163192486760401955554931445160137505740521734144;

J(5,1)= 0;
J(5,2)= cos(q1);
J(5,3)= cos(q1);
J(5,4)= (81129638414606686663546605165575*sin(q1 + q2 + q3))/162259276829213363391578010288128 - (81129638414606676728031405122553*sin(q2 - q1 + q3))/162259276829213363391578010288128 + (4967757600021511*cos(q1))/81129638414606681695789005144064;
J(5,5)= cos(q1 - q4)/2 + (403032377821159498335588895202304015643716683825*sin(q1 + q2 + q3))/13164036458569648337239753460458804039861886925068638906788872192 + (6582018229284823362555121087910479384599870772374890568949237809*sin(q1 - q2 - q3 + q4))/26328072917139296674479506920917608079723773850137277813577744384 - (403032377821159448978357750059338280708391237583*sin(q2 - q1 + q3))/13164036458569648337239753460458804039861886925068638906788872192 - (6582018229284824974684632372548374012493161295659483273165080625*sin(q1 + q2 + q3 + q4))/26328072917139296674479506920917608079723773850137277813577744384 + cos(q1 + q4)/2 + (24678615572571482867467662723121*cos(q1))/6582018229284824168619876730229402019930943462534319453394436096 + (6582018229284824168619876730229377341315370891051451985731712975*sin(q1 + q2 + q3 - q4))/26328072917139296674479506920917608079723773850137277813577744384 + (6582018229284824168619876730229377341315370891051451985731712975*sin(q2 - q1 + q3 + q4))/26328072917139296674479506920917608079723773850137277813577744384;
J(5,6)= (122597380068651197257713859414983140362437055831*cos(q1))/533996758980227520598755426542388028650676130589163192486760401955554931445160137505740521734144 + (4967757600021511*cos(q1)*cos(q4))/81129638414606681695789005144064 - (24678615572571482867467662723121*sin(q3)*((81129638414606676728031405122553*cos(q1 - q2))/2 - (81129638414606686663546605165575*cos(q1 + q2))/2))/533996758980227520598755426542388028650676130589163192486760401955554931445160137505740521734144 + (24678615572571482867467662723121*cos(q3)*((81129638414606676728031405122553*sin(q1 - q2))/2 + (81129638414606686663546605165575*sin(q1 + q2))/2))/533996758980227520598755426542388028650676130589163192486760401955554931445160137505740521734144 + cos(q5)*((81129638414606686663546605165575*sin(q1 + q2 + q3))/162259276829213363391578010288128 - (81129638414606676728031405122553*sin(q2 - q1 + q3))/162259276829213363391578010288128 + (4967757600021511*cos(q1))/81129638414606681695789005144064) + (4967757600021511*cos(q5)*((sin(q4)*(81129638414606686663546605165575*cos(q1 + q2 + q3) - 81129638414606676728031405122553*cos(q2 - q1 + q3)))/162259276829213363391578010288128 - cos(q1)*cos(q4) + (4967757600021511*cos(q4)*((81129638414606686663546605165575*sin(q1 + q2 + q3))/162259276829213363391578010288128 - (81129638414606676728031405122553*sin(q2 - q1 + q3))/162259276829213363391578010288128))/81129638414606681695789005144064))/81129638414606681695789005144064 + sin(q5)*(cos(q1)*sin(q4) - (4967757600021511*sin(q4)*((81129638414606686663546605165575*sin(q1 + q2 + q3))/162259276829213363391578010288128 - (81129638414606676728031405122553*sin(q2 - q1 + q3))/162259276829213363391578010288128))/81129638414606681695789005144064 + cos(q4)*((81129638414606686663546605165575*cos(q1 + q2 + q3))/162259276829213363391578010288128 - (81129638414606676728031405122553*cos(q2 - q1 + q3))/162259276829213363391578010288128)) - (4967757600021511*sin(q4)*((81129638414606686663546605165575*cos(q1 + q2 + q3))/162259276829213363391578010288128 - (81129638414606676728031405122553*cos(q2 - q1 + q3))/162259276829213363391578010288128))/81129638414606681695789005144064 - (24678615572571482867467662723121*cos(q4)*((81129638414606686663546605165575*sin(q1 + q2 + q3))/162259276829213363391578010288128 - (81129638414606676728031405122553*sin(q2 - q1 + q3))/162259276829213363391578010288128))/6582018229284824168619876730229402019930943462534319453394436096;

J(6,1)= 1;
J(6,2)=4967757600021511/81129638414606681695789005144064;
J(6,3)=4967757600021511/81129638414606681695789005144064;
J(6,4)=24678615572571482867467662723121/6582018229284824168619876730229402019930943462534319453394436096 - sin(q2 + q3);
J(6,5)=(81129638414606686663546605165575*sin(q2 + q3 + q4))/162259276829213363391578010288128 - (81129638414606676728031405122553*sin(q2 + q3 - q4))/162259276829213363391578010288128 - (4967757600021511*sin(q2 + q3))/81129638414606681695789005144064 + (4967757600021511*cos(q4))/81129638414606681695789005144064 + 122597380068651197257713859414983140362437055831/533996758980227520598755426542388028650676130589163192486760401955554931445160137505740521734144;
J(6,6)=(403032377821159448978357750059338280708391237583*cos(q4 - q5))/13164036458569648337239753460458804039861886925068638906788872192 + (403032377821159498335588895202304015643716683825*sin(q2 + q3 + q4))/13164036458569648337239753460458804039861886925068638906788872192 - sin(q2 + q3 + q5)/2 + (6582018229284824168619876730229377341315370891051451985731712975*sin(q2 + q3 - q4 - q5))/26328072917139296674479506920917608079723773850137277813577744384 - (403032377821159448978357750059338280708391237583*sin(q2 + q3 - q4))/13164036458569648337239753460458804039861886925068638906788872192 - sin(q2 + q3 - q5)/2 - (6582018229284824974684632372548374012493161295659483273165080625*sin(q2 + q3 + q4 + q5))/26328072917139296674479506920917608079723773850137277813577744384 - (403032377821159498335588895202304015643716683825*cos(q4 + q5))/13164036458569648337239753460458804039861886925068638906788872192 - (24678615572571482867467662723121*sin(q2 + q3))/6582018229284824168619876730229402019930943462534319453394436096 + (24678615572571482867467662723121*cos(q4))/6582018229284824168619876730229402019930943462534319453394436096 + (24678615572571482867467662723121*cos(q5))/6582018229284824168619876730229402019930943462534319453394436096 + (6582018229284824168619876730229377341315370891051451985731712975*sin(q2 + q3 + q4 - q5))/26328072917139296674479506920917608079723773850137277813577744384 - (6582018229284823362555121087910479384599870772374890568949237809*sin(q2 + q3 - q4 + q5))/26328072917139296674479506920917608079723773850137277813577744384 + 609034066578767699168763939638324732237239140958410949107980641/43322963970637732180912721627235682866194329302747133987038743447103457934462900359999600095377180907771737671271930809827721216;

d_ef = [dx dy dz d_alpha d_beta d_gamma ]';
 
% d_joint = inv(j_matrix)*d_ef;
d_joint = J\d_ef;
dq1=d_joint(1);
dq2=d_joint(2);
dq3=d_joint(3);
dq4=d_joint(4);
dq5=d_joint(5);
dq6=d_joint(6);

% output_joint_value =zeros(6,1);
% dt=0.001;
% output_joint_value(1) = dq1*dt + q1;
% output_joint_value(2) = dq2*dt + q2;
% output_joint_value(3) = dq3*dt + q3;
% output_joint_value(4) = dq4*dt + q4;
% output_joint_value(5) = dq5*dt + q5;
% output_joint_value(6) = dq6*dt + q6;

output_djoint_value =zeros(6,1);

output_djoint_value(1) = dq1;
output_djoint_value(2) = dq2;
output_djoint_value(3) = dq3;
output_djoint_value(4) = dq4;
output_djoint_value(5) = dq5;
output_djoint_value(6) = dq6;
%det_J 
det_J = det(J);
end
